simulink model "ASM_Traffic_MultiCore"  (R2026a)
settings: Solver=ode1  StartTime=SIM.tstart.v  StopTime=SIM.tend.v  FixedStep=SIM.StepSize.v
PostLoadFcn:
  | if any(exist('dsrtsu_mdlpostloadfcn', 'file') ~= 0), dsrtsu_mdlpostloadfcn('Execute', bdroot); end
  | try, asm_mdl_postloadfcn(bdroot, 'UpdateModel', 3600); catch, disp(lasterr); end,
InitFcn:
  | , if any(exist('rtifpga_mdlclblib', 'file') ~= 0), rtifpga_mdlclblib('Init', bdroot); end,
  | , if any(exist('dsmpb_private', 'file') ~= 0), dsmpb_private('dsmpb_mdlclblib', 'Init', bdroot); end,
model workspace (MAT data in the model file):
  asmReferencePath = [0 0.01 0.02 0.03 0.04 0.05 0.06 0.07 0.08 0.09 0.1 0.11 ... (350007 elements, 50001x7)]
  roadBounds : Simulink.Parameter (value not decoded)
  safetyAxes : Simulink.Parameter (value not decoded)
undefined symbols (not defined in the file): _to_, a0b2, ASM_BrakeHydraulics_DemoSystems, ASM_VehicleDynamics_DemoSystems, b98103fe8ad365046cd0, BrakeCircuit, controllerConfig, CPT, Crankshaft, DiscIntNeverNeededParam, dsmsi, FinalDriveAssembly, MDL, ModeSignals, mu, Pos_BrakePedal_Maneuver, rad, RefSignals, roadFamilyData, roadFamilyId, s_to_rpm, SIM, SoftECU, Suspension, Tire, Transmission
libraries: ASM_Traffic_lib x135, simulink x98, ASM_Utils_lib x77, ASM_VehicleDynamics_lib x70, ASM_Environment_lib x22, dsmpblib x20, dsmsilib x15, MDLD_Utils_lib x10, ASM_BrakeHydraulics_lib x3, sl_discontinuities x2
(part 25 of 65)

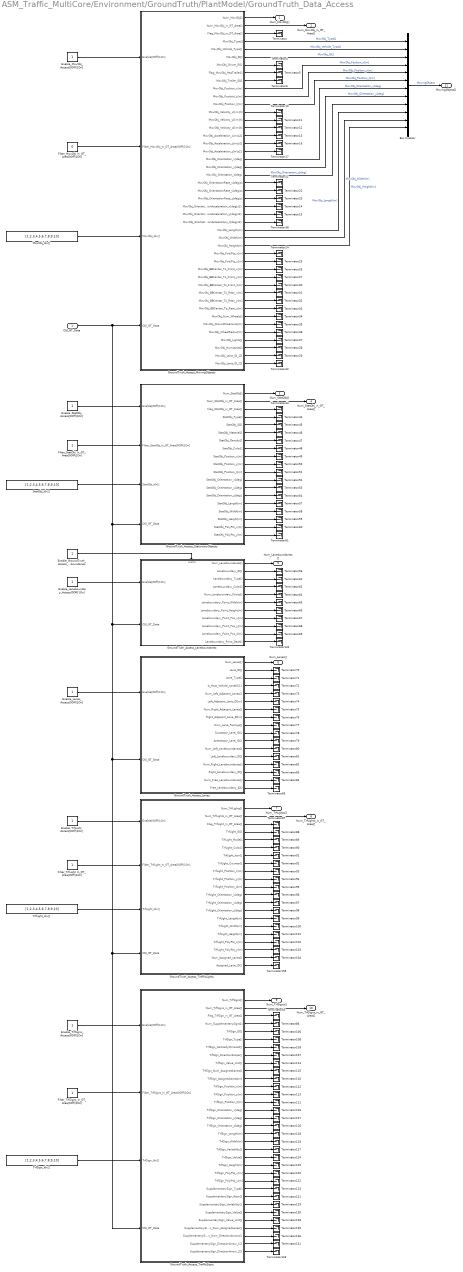
== system ASM_Traffic_MultiCore/Environment/GroundTruth/PlantModel/GroundTruth_Data_Access ==
  OSI_GT_Data : Inport
  Bus Creator : BusCreator  Inputs=12
  Enable_GroundTruth_Access_Laneboundaries : Constant
  Enable_Laneboundary_Access[0Off|1On] : Constant
  Enable_Lanes_Access[0Off|1On] : Constant
  Enable_MovObj_Access[0Off|1On] : Constant
  Enable_StatObj_Access[0Off|1On] : Constant
  Enable_TrfLight_Access[0Off|1On] : Constant
  Enable_TrfSigns_Access[0Off|1On] : Constant
  Filter_MovObj_In_GT_Area[0Off|1On] : Constant  Value=0
  Filter_StatObj_In_GT_Area[0Off|1On] : Constant
  Filter_TrfLight_In_GT_Area[0Off|1On] : Constant
  Filter_TrfSigns_In_GT_Area[0Off|1On] : Constant
  GroundTruth_Access_Laneboundaries : Subsystem
  GroundTruth_Access_Lanes : Subsystem
  GroundTruth_Access_MovingObjects : Subsystem
  GroundTruth_Access_StationaryObjects : Subsystem
  GroundTruth_Access_TrafficLights : Subsystem
  GroundTruth_Access_TrafficSigns : Subsystem
  MovObj_Idx[] : Constant  Value=[1,2,3,4,5,6,7,8,9,10]
  StatObj_Idx[] : Constant  Value=[1,2,3,4,5,6,7,8,9,10]
  Terminator{,4..6,10..17,21..38,42..133,135..136} (124 alike) : Terminator
  TrfLight_Idx[] : Constant  Value=[1,2,3,4,5,6,7,8,9,10]
  TrfSign_Idx[] : Constant  Value=[1,2,3,4,5,6,7,8,9,10]
  Num_MovObj[] : Outport  VectorParamsAs1DForOutWhenUnconnected=off
  Num_MovObj_in_GT_Area[] : Outport  Port=2  VectorParamsAs1DForOutWhenUnconnected=off
  Num_StatObj[] : Outport  Port=3  VectorParamsAs1DForOutWhenUnconnected=off
  Num_StatObj_in_GT_Area[] : Outport  Port=4  VectorParamsAs1DForOutWhenUnconnected=off
  Num_Laneboundaries[] : Outport  Port=5  VectorParamsAs1DForOutWhenUnconnected=off
  Num_Lanes[] : Outport  Port=6  VectorParamsAs1DForOutWhenUnconnected=off
  Num_TrfLights[] : Outport  Port=7  VectorParamsAs1DForOutWhenUnconnected=off
  Num_TrfLights_in_GT_Area[] : Outport  Port=8  VectorParamsAs1DForOutWhenUnconnected=off
  Num_TrfSigns[] : Outport  Port=9  VectorParamsAs1DForOutWhenUnconnected=off
  Num_TrfSigns_in_GT_Area[] : Outport  Port=10  VectorParamsAs1DForOutWhenUnconnected=off
  MovingObject[] : Outport  Port=11
  wires:
  Bus Creator/1 -> MovingObject[]/1  "MovingObject"
  GroundTruth_Access_Laneboundaries/11(Laneboundary_Point_Dash[]) -> Terminator132/1
  Enable_GroundTruth_Access_Laneboundaries/1 -> GroundTruth_Access_Laneboundaries/Enable
  GroundTruth_Access_MovingObjects/45(MovObj_Lane_ID_2[]) -> Terminator42/1
  GroundTruth_Access_MovingObjects/44(MovObj_Lane_ID_1[]) -> Terminator29/1
  GroundTruth_Access_MovingObjects/43(MovObj_NumLanes[]) -> Terminator28/1
  GroundTruth_Access_MovingObjects/42(MovObj_Lights[]) -> Terminator37/1
  GroundTruth_Access_MovingObjects/41(MovObj_WheelRadius[m]) -> Terminator36/1
  GroundTruth_Access_MovingObjects/40(MovObj_GroundClearance[m]) -> Terminator35/1
  GroundTruth_Access_MovingObjects/39(MovObj_Num_Wheels[]) -> Terminator34/1
  GroundTruth_Access_MovingObjects/38(MovObj_BBCenter_To_Rear_z[m]) -> Terminator33/1
  GroundTruth_Access_MovingObjects/37(MovObj_BBCenter_To_Rear_y[m]) -> Terminator32/1
  GroundTruth_Access_MovingObjects/36(MovObj_BBCenter_To_Rear_x[m]) -> Terminator31/1
  GroundTruth_Access_MovingObjects/35(MovObj_BBCenter_To_Front_z[m]) -> Terminator30/1
  GroundTruth_Access_MovingObjects/34(MovObj_BBCenter_To_Front_y[m]) -> Terminator27/1
  GroundTruth_Access_MovingObjects/33(MovObj_BBCenter_To_Front_x[m]) -> Terminator26/1
  GroundTruth_Access_MovingObjects/32(MovObj_PolyPts_y[m]) -> Terminator25/1
  GroundTruth_Access_MovingObjects/31(MovObj_PolyPts_x[m]) -> Terminator24/1
  GroundTruth_Access_MovingObjects/30(MovObj_Height[m]) -> Bus Creator/12  "MovObj_Height[m]"
  GroundTruth_Access_MovingObjects/29(MovObj_Width[m]) -> Bus Creator/11  "MovObj_Width[m]"
  GroundTruth_Access_MovingObjects/28(MovObj_Length[m]) -> Bus Creator/10  "MovObj_Length[m]"
  GroundTruth_Access_MovingObjects/27(MovObj_OrientationAcceleration_z[deg|s2]) -> Terminator38/1
  GroundTruth_Access_MovingObjects/26(MovObj_OrientationAcceleration_y[deg|s2]) -> Terminator15/1
  GroundTruth_Access_MovingObjects/25(MovObj_OrientationAcceleration_x[deg|s2]) -> Terminator14/1
  GroundTruth_Access_MovingObjects/24(MovObj_OrientationRate_z[deg|s]) -> Terminator23/1
  GroundTruth_Access_MovingObjects/23(MovObj_OrientationRate_y[deg|s]) -> Terminator22/1
  GroundTruth_Access_MovingObjects/22(MovObj_OrientationRate_x[deg|s]) -> Terminator21/1
  GroundTruth_Access_MovingObjects/21(MovObj_Orientation_z[deg]) -> Bus Creator/9  "MovObj_Orientation_z[deg]"
  GroundTruth_Access_MovingObjects/20(MovObj_Orientation_y[deg]) -> Bus Creator/8  "MovObj_Orientation_y[deg]"
  GroundTruth_Access_MovingObjects/19(MovObj_Orientation_x[deg]) -> Bus Creator/7  "MovObj_Orientation_x[deg]"
  GroundTruth_Access_MovingObjects/18(MovObj_Acceleration_z[m|s2]) -> Terminator17/1
  GroundTruth_Access_MovingObjects/17(MovObj_Acceleration_y[m|s2]) -> Terminator16/1
  GroundTruth_Access_MovingObjects/16(MovObj_Acceleration_x[m|s2]) -> Terminator13/1
  GroundTruth_Access_MovingObjects/15(MovObj_Velocity_z[km|h]) -> Terminator12/1
  GroundTruth_Access_MovingObjects/14(MovObj_Velocity_y[km|h]) -> Terminator11/1
  GroundTruth_Access_MovingObjects/13(MovObj_Velocity_x[km|h]) -> Terminator10/1
  GroundTruth_Access_MovingObjects/12(MovObj_Position_z[m]) -> Bus Creator/6  "MovObj_Position_z[m]"
  GroundTruth_Access_MovingObjects/11(MovObj_Position_y[m]) -> Bus Creator/5  "MovObj_Position_y[m]"
  GroundTruth_Access_MovingObjects/10(MovObj_Position_x[m]) -> Bus Creator/4  "MovObj_Position_x[m]"
  GroundTruth_Access_MovingObjects/9(MovObj_Trailer_ID[]) -> Terminator6/1
  GroundTruth_Access_MovingObjects/8(Flag_MovObj_HasTrailer[]) -> Terminator5/1
  GroundTruth_Access_MovingObjects/7(MovObj_Driver_ID[]) -> Terminator4/1
  GroundTruth_Access_MovingObjects/6(MovObj_ID[]) -> Bus Creator/3  "MovObj_ID[]"
  GroundTruth_Access_MovingObjects/5(MovObj_Vehicle_Type[]) -> Bus Creator/2  "MovObj_Vehicle_Type[]"
  GroundTruth_Access_MovingObjects/4(MovObj_Type[]) -> Bus Creator/1  "MovObj_Type[]"
  GroundTruth_Access_MovingObjects/3(Flag_MovObj_in_GT_Area[]) -> Terminator/1
  GroundTruth_Access_MovingObjects/2(Num_MovObj_in_GT_Area[]) -> Num_MovObj_in_GT_Area[]/1
  GroundTruth_Access_MovingObjects/1(Num_MovObj[]) -> Num_MovObj[]/1
  OSI_GT_Data/1 -> GroundTruth_Access_StationaryObjects/4(OSI_GT_Data), GroundTruth_Access_TrafficSigns/4(OSI_GT_Data), GroundTruth_Access_TrafficLights/4(OSI_GT_Data), GroundTruth_Access_Lanes/2(OSI_GT_Data), GroundTruth_Access_Laneboundaries/2(OSI_GT_Data), GroundTruth_Access_MovingObjects/4(OSI_GT_Data)
  MovObj_Idx[]/1 -> GroundTruth_Access_MovingObjects/3(MovObj_Idx[])
  Filter_MovObj_In_GT_Area[0Off|1On]/1 -> GroundTruth_Access_MovingObjects/2(Filter_MovObj_In_GT_Area[0Off|1On])
  Enable_MovObj_Access[0Off|1On]/1 -> GroundTruth_Access_MovingObjects/1(Enable[0Off|1On])
  GroundTruth_Access_StationaryObjects/2(Num_StatObj_in_GT_Area[]) -> Num_StatObj_in_GT_Area[]/1
  Enable_StatObj_Access[0Off|1On]/1 -> GroundTruth_Access_StationaryObjects/1(Enable[0Off|1On])
  Filter_StatObj_In_GT_Area[0Off|1On]/1 -> GroundTruth_Access_StationaryObjects/2(Filter_StatObj_In_GT_Area[0Off|1On])
  StatObj_Idx[]/1 -> GroundTruth_Access_StationaryObjects/3(StatObj_Idx[])
  GroundTruth_Access_Laneboundaries/1(Num_Laneboundaries[]) -> Num_Laneboundaries[]/1
  GroundTruth_Access_Laneboundaries/2(Laneboundary_ID[]) -> Terminator56/1
  GroundTruth_Access_Laneboundaries/3(Laneboundary_Type[]) -> Terminator62/1
  GroundTruth_Access_Laneboundaries/4(Laneboundary_Color[]) -> Terminator63/1
  GroundTruth_Access_Laneboundaries/5(Num_Laneboundary_Points[]) -> Terminator64/1
  GroundTruth_Access_Laneboundaries/6(Laneboundary_Point_Width[m]) -> Terminator65/1
  GroundTruth_Access_Laneboundaries/7(Laneboundary_Point_Height[m]) -> Terminator66/1
  GroundTruth_Access_Laneboundaries/8(Laneboundary_Point_Pos_x[m]) -> Terminator67/1
  GroundTruth_Access_Laneboundaries/9(Laneboundary_Point_Pos_y[m]) -> Terminator68/1
  GroundTruth_Access_Laneboundaries/10(Laneboundary_Point_Pos_z[m]) -> Terminator69/1
  Enable_Laneboundary_Access[0Off|1On]/1 -> GroundTruth_Access_Laneboundaries/1(Enable[0Off|1On])
  GroundTruth_Access_Lanes/1(Num_Lanes[]) -> Num_Lanes[]/1
  GroundTruth_Access_Lanes/2(Lane_ID[]) -> Terminator70/1
  GroundTruth_Access_Lanes/3(Lane_Type[]) -> Terminator71/1
  GroundTruth_Access_Lanes/4(Is_Host_Vehicle_Lane[0|1]) -> Terminator72/1
  GroundTruth_Access_Lanes/5(Num_Left_Adjacent_Lanes[]) -> Terminator73/1
  GroundTruth_Access_Lanes/6(Left_Adjacent_Lane_ID[m]) -> Terminator74/1
  GroundTruth_Access_Lanes/7(Num_Right_Adjacent_Lanes[]) -> Terminator75/1
  GroundTruth_Access_Lanes/8(Right_Adjacent_Lane_ID[m]) -> Terminator76/1
  GroundTruth_Access_Lanes/9(Num_Lane_Pairings[]) -> Terminator77/1
  GroundTruth_Access_Lanes/10(Successor_Lane_ID[]) -> Terminator78/1
  GroundTruth_Access_Lanes/11(Antecessor_Lane_ID[]) -> Terminator79/1
  GroundTruth_Access_Lanes/12(Num_Left_Laneboundaries[]) -> Terminator80/1
  GroundTruth_Access_Lanes/13(Left_Laneboundary_ID[]) -> Terminator81/1
  GroundTruth_Access_Lanes/14(Num_Right_Laneboundaries[]) -> Terminator82/1
  GroundTruth_Access_Lanes/15(Right_Laneboundary_ID[]) -> Terminator83/1
  GroundTruth_Access_Lanes/16(Num_Free_Laneboundaries[]) -> Terminator84/1
  GroundTruth_Access_Lanes/17(Free_Laneboundary_ID[]) -> Terminator85/1
  Enable_Lanes_Access[0Off|1On]/1 -> GroundTruth_Access_Lanes/1(Enable[0Off|1On])
  GroundTruth_Access_TrafficLights/2(Num_TrfLights_in_GT_Area[]) -> Num_TrfLights_in_GT_Area[]/1
  GroundTruth_Access_TrafficLights/1(Num_TrfLights[]) -> Num_TrfLights[]/1
  GroundTruth_Access_TrafficLights/3(Flag_TrfLight_in_GT_Area[]) -> Terminator87/1
  GroundTruth_Access_TrafficLights/4(TrfLight_ID[]) -> Terminator88/1
  GroundTruth_Access_TrafficLights/5(TrfLight_Mode[]) -> Terminator89/1
  GroundTruth_Access_TrafficLights/6(TrfLight_Color[]) -> Terminator90/1
  GroundTruth_Access_TrafficLights/7(TrfLight_Icon[]) -> Terminator91/1
  GroundTruth_Access_TrafficLights/8(TrfLight_Counter[]) -> Terminator92/1
  GroundTruth_Access_TrafficLights/9(TrfLight_Position_x[m]) -> Terminator93/1
  GroundTruth_Access_TrafficLights/10(TrfLight_Position_y[m]) -> Terminator94/1
  GroundTruth_Access_TrafficLights/11(TrfLight_Position_z[m]) -> Terminator95/1
  GroundTruth_Access_TrafficLights/12(TrfLight_Orientation_x[deg]) -> Terminator96/1
  GroundTruth_Access_TrafficLights/13(TrfLight_Orientation_y[deg]) -> Terminator97/1
  GroundTruth_Access_TrafficLights/14(TrfLight_Orientation_z[deg]) -> Terminator98/1
  GroundTruth_Access_TrafficLights/15(TrfLight_Length[m]) -> Terminator99/1
  GroundTruth_Access_TrafficLights/16(TrfLight_Width[m]) -> Terminator100/1
  GroundTruth_Access_TrafficLights/17(TrfLight_Height[m]) -> Terminator101/1
  GroundTruth_Access_TrafficLights/18(TrfLight_PolyPts_x[m]) -> Terminator102/1
  GroundTruth_Access_TrafficLights/19(TrfLight_PolyPts_y[m]) -> Terminator103/1
  GroundTruth_Access_TrafficLights/20(Num_Assigned_Lanes[]) -> Terminator104/1
  GroundTruth_Access_TrafficLights/21(Assigned_Lane_ID[]) -> Terminator105/1
  Enable_TrfLight_Access[0Off|1On]/1 -> GroundTruth_Access_TrafficLights/1(Enable[0Off|1On])
  Filter_TrfLight_In_GT_Area[0Off|1On]/1 -> GroundTruth_Access_TrafficLights/2(Filter_TrfLight_In_GT_Area[0Off|1On])
  TrfLight_Idx[]/1 -> GroundTruth_Access_TrafficLights/3(TrfLight_Idx[])
  GroundTruth_Access_TrafficSigns/3(Flag_TrfSign_in_GT_Area[]) -> Terminator55/1
  GroundTruth_Access_TrafficSigns/4(Num_SupplementarySigns[]) -> Terminator86/1
  GroundTruth_Access_TrafficSigns/5(TrfSign_ID[]) -> Terminator106/1
  GroundTruth_Access_TrafficSigns/6(TrfSign_Type[]) -> Terminator108/1
  GroundTruth_Access_TrafficSigns/7(TrfSign_VerticallyMirrored[]) -> Terminator109/1
  GroundTruth_Access_TrafficSigns/8(TrfSign_DirectionScope[]) -> Terminator107/1
  GroundTruth_Access_TrafficSigns/14(TrfSign_Position_z[m]) -> Terminator111/1
  GroundTruth_Access_TrafficSigns/13(TrfSign_Position_y[m]) -> Terminator113/1
  GroundTruth_Access_TrafficSigns/12(TrfSign_Position_x[m]) -> Terminator112/1
  GroundTruth_Access_TrafficSigns/11(TrfSign_AssignedLanes[m]) -> Terminator110/1
  GroundTruth_Access_TrafficSigns/10(TrfSign_Num_AssignedLanes[]) -> Terminator115/1
  GroundTruth_Access_TrafficSigns/9(TrfSign_Value_Unit[]) -> Terminator114/1
  GroundTruth_Access_TrafficSigns/21(TrfSign_Value[]) -> Terminator124/1
  GroundTruth_Access_TrafficSigns/22(TrfSign_Height[m]) -> Terminator125/1
  GroundTruth_Access_TrafficSigns/23(TrfSign_PolyPts_x[m]) -> Terminator120/1
  GroundTruth_Access_TrafficSigns/24(TrfSign_PolyPts_y[m]) -> Terminator122/1
  GroundTruth_Access_TrafficSigns/25(SupplementarySign_Type[]) -> Terminator123/1
  GroundTruth_Access_TrafficSigns/26(SupplementarySign_Actor[]) -> Terminator121/1
  GroundTruth_Access_TrafficSigns/20(TrfSign_Variability[]) -> Terminator117/1
  GroundTruth_Access_TrafficSigns/19(TrfSign_Width[m]) -> Terminator119/1
  GroundTruth_Access_TrafficSigns/18(TrfSign_Length[m]) -> Terminator118/1
  GroundTruth_Access_TrafficSigns/17(TrfSign_Orientation_z[deg]) -> Terminator116/1
  GroundTruth_Access_TrafficSigns/16(TrfSign_Orientation_y[deg]) -> Terminator127/1
  GroundTruth_Access_TrafficSigns/15(TrfSign_Orientation_x[deg]) -> Terminator126/1
  GroundTruth_Access_TrafficSigns/27(SupplementarySign_Variability[]) -> Terminator129/1
  GroundTruth_Access_TrafficSigns/28(SupplementarySign_Value[]) -> Terminator130/1
  GroundTruth_Access_TrafficSigns/29(SupplementarySign_Value_Unit[]) -> Terminator128/1
  GroundTruth_Access_TrafficSigns/33(SupplementarySign_DirectionArrow_2[]) -> Terminator133/1
  GroundTruth_Access_TrafficSigns/32(SupplementarySign_DirectionArrow_1[]) -> Terminator131/1
  GroundTruth_Access_TrafficSigns/31(SupplementarySign_Num_DirectionArrows[]) -> Terminator136/1
  GroundTruth_Access_TrafficSigns/30(SupplementarySign_Num_AssignedLanes[]) -> Terminator135/1
  Enable_TrfSigns_Access[0Off|1On]/1 -> GroundTruth_Access_TrafficSigns/1(Enable[0Off|1On])
  Filter_TrfSigns_In_GT_Area[0Off|1On]/1 -> GroundTruth_Access_TrafficSigns/2(Filter_TrfSigns_In_GT_Area[0Off|1On])
  TrfSign_Idx[]/1 -> GroundTruth_Access_TrafficSigns/3(TrfSign_Idx[])
  GroundTruth_Access_TrafficSigns/1(Num_TrfSigns[]) -> Num_TrfSigns[]/1
  GroundTruth_Access_TrafficSigns/2(Num_TrfSigns_in_GT_Area[]) -> Num_TrfSigns_in_GT_Area[]/1
  GroundTruth_Access_StationaryObjects/11(StatObj_Position_z[m]) -> Terminator51/1
  GroundTruth_Access_StationaryObjects/18(StatObj_PolyPts_x[m]) -> Terminator60/1
  GroundTruth_Access_StationaryObjects/4(StatObj_Type[]) -> Terminator44/1
  GroundTruth_Access_StationaryObjects/12(StatObj_Orientation_x[deg]) -> Terminator52/1
  GroundTruth_Access_StationaryObjects/15(StatObj_Length[m]) -> Terminator57/1
  GroundTruth_Access_StationaryObjects/14(StatObj_Orientation_z[deg]) -> Terminator54/1
  GroundTruth_Access_StationaryObjects/8(StatObj_Color[]) -> Terminator48/1
  GroundTruth_Access_StationaryObjects/3(Flag_StatObj_in_GT_Area[]) -> Terminator43/1
  GroundTruth_Access_StationaryObjects/10(StatObj_Position_y[m]) -> Terminator50/1
  GroundTruth_Access_StationaryObjects/7(StatObj_Density[]) -> Terminator47/1
  GroundTruth_Access_StationaryObjects/9(StatObj_Position_x[m]) -> Terminator49/1
  GroundTruth_Access_StationaryObjects/6(StatObj_Material[]) -> Terminator46/1
  GroundTruth_Access_StationaryObjects/13(StatObj_Orientation_y[deg]) -> Terminator53/1
  GroundTruth_Access_StationaryObjects/16(StatObj_Width[m]) -> Terminator58/1
  GroundTruth_Access_StationaryObjects/19(StatObj_PolyPts_y[m]) -> Terminator61/1
  GroundTruth_Access_StationaryObjects/17(StatObj_Height[m]) -> Terminator59/1
  GroundTruth_Access_StationaryObjects/5(StatObj_ID[]) -> Terminator45/1
  GroundTruth_Access_StationaryObjects/1(Num_StatObj[]) -> Num_StatObj[]/1

== system ASM_Traffic_MultiCore/Environment/GroundTruth/PlantModel/HostVehicle_Data_Access ==
  OSI_HV_Data : Inport
  Enable_HostVehicle_Data_Access[0Off|1On] : Constant
  HostVehicle_Data_Access : Subsystem
  Terminator{,1..23} (24 alike) : Terminator
  wires:
  HostVehicle_Data_Access/5(HV_Position_BB[x;y;z][m]) -> Terminator4/1
  HostVehicle_Data_Access/6(HV_Velocity_BB[x;y;z][m|s]) -> Terminator5/1
  HostVehicle_Data_Access/3(HV_ID[]) -> Terminator2/1
  HostVehicle_Data_Access/4(HV_Pos_BrakePedal[0_1]) -> Terminator3/1
  HostVehicle_Data_Access/2(Time_Stamp_Nanos[ns]) -> Terminator1/1
  Enable_HostVehicle_Data_Access[0Off|1On]/1 -> HostVehicle_Data_Access/1(Enable[0Off|1On])
  OSI_HV_Data/1 -> HostVehicle_Data_Access/2(OSI_HV_Data)
  HostVehicle_Data_Access/1(Time_Stamp_Seconds[s]) -> Terminator/1
  HostVehicle_Data_Access/7(HV_Acceleration_BB[x;y;z][m|s2]) -> Terminator6/1
  HostVehicle_Data_Access/8(HV_Orientation_BB[x;y;z][rad]) -> Terminator7/1
  HostVehicle_Data_Access/9(HV_Current_Curvature[1|m]) -> Terminator8/1
  HostVehicle_Data_Access/10(HV_Steering_Angle[rad]) -> Terminator9/1
  HostVehicle_Data_Access/11(HV_Steering_Angle_dt[rad|s]) -> Terminator10/1
  HostVehicle_Data_Access/12(HV_Steering_Torque[Nm]) -> Terminator11/1
  HostVehicle_Data_Access/13(HV_Pos_AccPedal[0_1]) -> Terminator12/1
  HostVehicle_Data_Access/14(HV_Pos_ClutchPedal[0_1]) -> Terminator13/1
  HostVehicle_Data_Access/15(HV_Gear[]) -> Terminator14/1
  HostVehicle_Data_Access/16(HV_Type_Engine[]) -> Terminator15/1
  HostVehicle_Data_Access/17(HV_n_Engine[rpm]) -> Terminator16/1
  HostVehicle_Data_Access/18(HV_Trq_Engine[Nm]) -> Terminator17/1
  HostVehicle_Data_Access/19(HV_Vehicle_Weight[kg]) -> Terminator18/1
  HostVehicle_Data_Access/20(HV_Vehicle_Operating_State[]) -> Terminator19/1
  HostVehicle_Data_Access/21(HV_WheelData_Axle_Idx[]) -> Terminator20/1
  HostVehicle_Data_Access/22(HV_WheelData_Wheel_Idx[]) -> Terminator21/1
  HostVehicle_Data_Access/23(HV_WheelData_Wheel_Speed[rad|s]) -> Terminator22/1
  HostVehicle_Data_Access/24(HV_WheelData_Wheel_Slip[]) -> Terminator23/1

== system ASM_Traffic_MultiCore/Environment/GroundTruth/PlantModel/ObjectDataStreams ==
  In : Inport
  Bus Selector14 : BusSelector  OutputSignals=DataStream_1[].DataStream_1[],DataStream_2[].DataStream_2[],DataStream_3[].DataStream_3[],DataStream_4[].DataStream_4[],DataStream_5[].DataStream_5[],DataStream_6[].DataStream_6[],DataStream_7[].DataStream_7[],DataStream_8[].DataStream_8[]
  Mux : Mux  Inputs=8
  Objects_DataStreams[] : Outport  VectorParamsAs1DForOutWhenUnconnected=off
  wires:
  Mux/1 -> Objects_DataStreams[]/1
  Bus Selector14/7 -> Mux/7  "<DataStream_7[]>"
  Bus Selector14/8 -> Mux/8  "<DataStream_8[]>"
  Bus Selector14/3 -> Mux/3  "<DataStream_3[]>"
  Bus Selector14/6 -> Mux/6  "<DataStream_6[]>"
  Bus Selector14/4 -> Mux/4  "<DataStream_4[]>"
  Bus Selector14/1 -> Mux/1  "<DataStream_1[]>"
  Bus Selector14/5 -> Mux/5  "<DataStream_5[]>"
  In/1 -> Bus Selector14/1
  Bus Selector14/2 -> Mux/2  "<DataStream_2[]>"

== system ASM_Traffic_MultiCore/Environment/GroundTruth/PlantModel/Running_Maneuver ==
  ManeuverState[] : Inport
  Brake : RelationalOperator  Operator===  OutDataTypeStr=boolean  InputSameDT=off
  Constant : Constant  Value=3
  Constant1 : Constant  Value=4
  Data Type Conversion : DataTypeConversion  OutDataTypeStr=double  SaturateOnIntegerOverflow=off  RndMeth=Floor
  Logical Operator : Logic  Operator=OR  AllPortsSameDT=off  OutDataTypeStr=boolean
  Run : RelationalOperator  Operator===  OutDataTypeStr=boolean  InputSameDT=off
  EnableRun[0Off|1On] : Outport  VectorParamsAs1DForOutWhenUnconnected=off
  wires:
  Run/1 -> Logical Operator/1
  ManeuverState[]/1 -> Brake/1, Run/1
  Constant1/1 -> Brake/2
  Logical Operator/1 -> Data Type Conversion/1
  Constant/1 -> Run/2
  Brake/1 -> Logical Operator/2
  Data Type Conversion/1 -> EnableRun[0Off|1On]/1

== system ASM_Traffic_MultiCore/Environment/GroundTruth/PlantModel/TrafficLight_Counter ==
  In : Inport
  Bus Selector14 : BusSelector  OutputSignals=TrafficLight_Counter_1[].TrafficLight_Counter_1[],TrafficLight_Counter_2.TrafficLight_Counter_2[],TrafficLight_Counter_3.TrafficLight_Counter_3[],TrafficLight_Counter_4[].TrafficLight_Counter_4[]
  Mux2 : Mux
  TrafficLight_Counter[] : Outport  VectorParamsAs1DForOutWhenUnconnected=off
  wires:
  Bus Selector14/1 -> Mux2/1  "<TrafficLight_Counter_1[]>"
  In/1 -> Bus Selector14/1
  Bus Selector14/3 -> Mux2/3  "<TrafficLight_Counter_3[]>"
  Bus Selector14/2 -> Mux2/2  "<TrafficLight_Counter_2[]>"
  Bus Selector14/4 -> Mux2/4  "<TrafficLight_Counter_4[]>"
  Mux2/1 -> TrafficLight_Counter[]/1

== system ASM_Traffic_MultiCore/Environment/GroundTruth/PlantModel/VehicleBasics ==
  In : Inport
  OSIGroundTruth : Inport  Port=2
  Bus Selector : BusSelector  OutputSignals=Interface_In.ExternalModel.m_TotalVehicle[kg],Interface_In.ExternalModel.State_StartButton[-2|-1|0|1|2|3]
  Bus Selector1 : BusSelector  OutputSignals=HostVehicle_Data_VehicleBasics[].Mode_OperatingState[1Stim|2Int],HostVehicle_Data_VehicleBasics[].Stim_OperatingState[]
  Multiport Switch : MultiPortSwitch  Inputs=2  SaturateOnIntegerOverflow=off  InputSameDT=off
  StartButton_Mapping : Subsystem
  m_TotalVehicle[kg] : Outport  VectorParamsAs1DForOutWhenUnconnected=off
  OperatingState[] : Outport  Port=2  VectorParamsAs1DForOutWhenUnconnected=off
  wires:
  Multiport Switch/1 -> OperatingState[]/1  "OperatingState[]"
  Bus Selector1/2 -> Multiport Switch/2  "<Stim_OperatingState[]>"
  Bus Selector1/1 -> Multiport Switch/1  "<Mode_OperatingState[1Stim|2Int]>"
  OSIGroundTruth/1 -> Bus Selector1/1
  In/1 -> Bus Selector/1
  Bus Selector/1 -> m_TotalVehicle[kg]/1  "<m_TotalVehicle[kg]>"
  Bus Selector/2 -> StartButton_Mapping/1(State_StartButton[-2|-1|0|1|2|3])  "<State_StartButton[-2|-1|0|1|2|3]>"
  StartButton_Mapping/1(OperatingState[]) -> Multiport Switch/3

== system ASM_Traffic_MultiCore/Environment/GroundTruth/PlantModel/VehicleBrakeSystem ==
  In : Inport
  Bus Selector25 : BusSelector  OutputSignals=Interface_In.ExternalModel.Pos_BrakePedal[%]
  Gain : Gain  Gain=1/100
  Pos_BrakePedal[0_1] : Outport
  wires:
  Bus Selector25/1 -> Gain/1  "<Pos_BrakePedal[%]>"
  In/1 -> Bus Selector25/1
  Gain/1 -> Pos_BrakePedal[0_1]/1

== system ASM_Traffic_MultiCore/Environment/GroundTruth/PlantModel/VehicleLocalization ==
  In : Inport
  Bus Selector : BusSelector  OutputSignals=Longitude[deg],Latitude[deg]
  Bus Selector10 : BusSelector  OutputSignals=Maneuver.Plant.ManeuverScheduler.Parameters.Object_Type_ID[]
  Bus Selector2 : BusSelector  OutputSignals=Interface_In.ExternalModel.Pos_Vehicle_CoorSys_E[x;y;z][m]
  Bus Selector22 : BusSelector  OutputSignals=Road.Plant.UserSignals_Customized
  Bus Selector3 : BusSelector  OutputSignals=Object_Properties_Box.PosVec_x_CenterPnt_Object[m],Object_Properties_Box.PosVec_y_CenterPnt_Object[m],Object_Properties_Box.PosVec_z_CenterPnt_Object[m]
  Bus Selector4 : BusSelector  OutputSignals=Interface_In.ExternalModel.Angle_Vehicle_CoorSys_E[x;y;z][deg]
  Bus Selector5 : BusSelector  OutputSignals=Traffic.Plant.ObjectParameters.TrafficObjects.TrafficObject_Type_Data[]
  COORDINATE_TRANSFORMATION_B_TO_A : ASM_Utils_lib/MatrixOperations/COORDINATE_TRANSFORMATION_B_TO_A  ASMLibrary2Check=ASM_Traffic_lib
  ChangeLabel : Subsystem
      mask Display: disp('')
  Demux : Demux  Outputs=3
  Demux1 : Demux  Outputs=3
  GPS_POSITION : ASM_Environment_lib/Environment/Road/GPS_POSITION  Tag=ASM_SUBCOMPONENT  ASMProperties=struct('Name','GPS_POSITION','Version','3.0','Library','ASM_Environment_lib')  ASMInstanceName=GPS_Position  ASMInstanceID=2
      settings: AttributesFormatString=Instance Name: %<ASMInstanceName>\nInstance ID: %<ASMInstanceID>
  Mux : Mux  Inputs=3
  OBJECT_PROPERTIES_BOX : ASM_Traffic_lib/Objects/OBJECT_PROPERTIES_BOX  ASMProperties=struct('Name','OBJECT_PROPERTIES_BOX','Version','2.0','Library','ASM_Traffic_lib')  ASMInstanceName=object_properties_box  ASMInstanceID=1
  Terminator : Terminator
  Terminator1 : Terminator
  Pos_Veh_BoundingBox_GPS[Long;Lat;Alt][deg;deg;m] : Outport
  wires:
  Bus Selector22/1 -> GPS_POSITION/1  "<UserSignals_Customized>"
  GPS_POSITION/1 -> Terminator/1
  GPS_POSITION/2 -> Bus Selector/1
  Bus Selector/1 -> Mux/1  "<Longitude[deg]>"
  Bus Selector/2 -> Mux/2  "<Latitude[deg]>"
  Mux/1 -> Pos_Veh_BoundingBox_GPS[Long;Lat;Alt][deg;deg;m]/1
  Bus Selector10/1 -> OBJECT_PROPERTIES_BOX/1  "<Object_Type_ID[]>"
  In/1 -> Bus Selector4/1, Bus Selector5/1, Bus Selector10/1, Bus Selector2/1, Bus Selector22/1
  Bus Selector5/1 -> OBJECT_PROPERTIES_BOX/2  "<TrafficObject_Type_Data[]>"
  OBJECT_PROPERTIES_BOX/1 -> Terminator1/1
  Bus Selector2/1 -> Demux/1  "<Pos_Vehicle_CoorSys_E[x;y;z][m]>"
  Demux/1 -> COORDINATE_TRANSFORMATION_B_TO_A/1
  Demux/2 -> COORDINATE_TRANSFORMATION_B_TO_A/2
  Demux/3 -> COORDINATE_TRANSFORMATION_B_TO_A/3
  Bus Selector3/2 -> COORDINATE_TRANSFORMATION_B_TO_A/5  "<PosVec_y_CenterPnt_Object[m]>"
  Bus Selector3/1 -> COORDINATE_TRANSFORMATION_B_TO_A/4  "<PosVec_x_CenterPnt_Object[m]>"
  Bus Selector3/3 -> COORDINATE_TRANSFORMATION_B_TO_A/6  "<PosVec_z_CenterPnt_Object[m]>"
  OBJECT_PROPERTIES_BOX/2 -> Bus Selector3/1
  Demux1/1 -> COORDINATE_TRANSFORMATION_B_TO_A/7
  Demux1/2 -> COORDINATE_TRANSFORMATION_B_TO_A/8
  Demux1/3 -> COORDINATE_TRANSFORMATION_B_TO_A/9
  COORDINATE_TRANSFORMATION_B_TO_A/3 -> ChangeLabel/1(In1)  "Pos_z_CoorSysE[m]"
  COORDINATE_TRANSFORMATION_B_TO_A/1 -> GPS_POSITION/2  "Pos_x_CoorSysE[m]"
  COORDINATE_TRANSFORMATION_B_TO_A/2 -> GPS_POSITION/3  "Pos_y_CoorSysE[m]"
  Bus Selector4/1 -> Demux1/1  "<Angle_Vehicle_CoorSys_E[x;y;z][deg]>"
  ChangeLabel/1(Out1) -> Mux/3  "Altitude[m]"

== system ASM_Traffic_MultiCore/Environment/GroundTruth/PlantModel/VehiclePowertrain ==
  In : Inport
  Bus Selector : BusSelector  OutputSignals=Interface_In.ExternalModel.Pos_AccPedal[%],Interface_In.ExternalModel.Pos_ClutchPedal[%],Interface_In.ExternalModel.Gear[],Interface_In.ExternalModel.n_Engine_1[rpm],Interface_In.ExternalModel.n_Engine_2[rpm],Interface_In.ExternalModel.Type_Engine_1[0Unkown|1Other|2Otto|3Diesel|4Electric],Interface_In.ExternalModel.Type_Engine_2[0Unkown|1Other|2Otto|3Diesel|4Electric],Interface_In.ExternalModel.Trq_Engine_1[Nm],Interface_In.ExternalModel.Trq_Engine_2[Nm]
  Gain : Gain  Gain=1/100
  Gain1 : Gain  Gain=1/100
  Mux : Mux  Inputs=2
  Mux1 : Mux  Inputs=2
  Mux2 : Mux  Inputs=2
  Pos_AccPedal[0_1] : Outport  VectorParamsAs1DForOutWhenUnconnected=off
  Pos_ClutchPedal[0_1] : Outport  Port=2  VectorParamsAs1DForOutWhenUnconnected=off
  Gear[] : Outport  Port=3  VectorParamsAs1DForOutWhenUnconnected=off
  n_Engine[rpm] : Outport  Port=4  VectorParamsAs1DForOutWhenUnconnected=off
  Type_Engine[0Unkown|1Other|2Otto|3Diesel|4Electric] : Outport  Port=5  VectorParamsAs1DForOutWhenUnconnected=off
  Trq_Engine[Nm] : Outport  Port=6  VectorParamsAs1DForOutWhenUnconnected=off
  wires:
  Bus Selector/3 -> Gear[]/1  "<Gear[]>"
  Bus Selector/4 -> Mux/1  "<n_Engine_1[rpm]>"
  Bus Selector/2 -> Gain1/1  "<Pos_ClutchPedal[%]>"
  In/1 -> Bus Selector/1
  Bus Selector/1 -> Gain/1  "<Pos_AccPedal[%]>"
  Mux/1 -> n_Engine[rpm]/1
  Bus Selector/5 -> Mux/2  "<n_Engine_2[rpm]>"
  Bus Selector/6 -> Mux1/1  "<Type_Engine_1[0Unkown|1Other|2Otto|3Diesel|4Electric]>"
  Bus Selector/7 -> Mux1/2  "<Type_Engine_2[0Unkown|1Other|2Otto|3Diesel|4Electric]>"
  Bus Selector/8 -> Mux2/1  "<Trq_Engine_1[Nm]>"
  Bus Selector/9 -> Mux2/2  "<Trq_Engine_2[Nm]>"
  Mux1/1 -> Type_Engine[0Unkown|1Other|2Otto|3Diesel|4Electric]/1
  Mux2/1 -> Trq_Engine[Nm]/1
  Gain/1 -> Pos_AccPedal[0_1]/1
  Gain1/1 -> Pos_ClutchPedal[0_1]/1

== system ASM_Traffic_MultiCore/Environment/GroundTruth/PlantModel/VehicleSteering ==
  In : Inport
  Bus Selector24 : BusSelector  OutputSignals=Interface_In.ExternalModel.Angle_SteeringWheel_SteeringSystem[deg],Interface_In.ExternalModel.Angle_SteeringWheel_dt_SteeringSystem[deg|s],Interface_In.ExternalModel.Trq_SteeringWheel_SteeringSystem[Nm]
  UnitConversion : ASM_Utils_lib/UnitConversion/UnitConversion  Selection=deg_to_rad
  UnitConversion1 : ASM_Utils_lib/UnitConversion/UnitConversion  Selection=deg_to_rad
  Angle_SteeringWheel_SteeringSystem[rad] : Outport  VectorParamsAs1DForOutWhenUnconnected=off
  Angle_SteeringWheel_dt_SteeringSystem[rad|s] : Outport  Port=2  VectorParamsAs1DForOutWhenUnconnected=off
  Trq_SteeringWheel_SteeringSystem[Nm] : Outport  Port=3  VectorParamsAs1DForOutWhenUnconnected=off
  wires:
  In/1 -> Bus Selector24/1
  Bus Selector24/1 -> UnitConversion/1  "<Angle_SteeringWheel_SteeringSystem[deg]>"
  Bus Selector24/2 -> UnitConversion1/1  "<Angle_SteeringWheel_dt_SteeringSystem[deg|s]>"
  Bus Selector24/3 -> Trq_SteeringWheel_SteeringSystem[Nm]/1  "<Trq_SteeringWheel_SteeringSystem[Nm]>"
  UnitConversion/1 -> Angle_SteeringWheel_SteeringSystem[rad]/1
  UnitConversion1/1 -> Angle_SteeringWheel_dt_SteeringSystem[rad|s]/1

== system ASM_Traffic_MultiCore/Environment/GroundTruth/PlantModel/VehicleWheels ==
  In : Inport
  OSIGroundTruth : Inport  Port=2
  Bus Selector1 : BusSelector  OutputSignals=HostVehicle_Data_VehicleWheels[].Axle_Idx[],HostVehicle_Data_VehicleWheels[].Wheel_Idx[]
  Bus Selector37 : BusSelector  OutputSignals=Interface_In.ExternalModel.omega_Wheel[rad|s],Interface_In.ExternalModel.Slip_x_Wheel[]
  Axle_Idx[] : Outport  VectorParamsAs1DForOutWhenUnconnected=off
  Wheel_Idx[] : Outport  Port=2  VectorParamsAs1DForOutWhenUnconnected=off
  omega_Wheel[rad|s] : Outport  Port=3  VectorParamsAs1DForOutWhenUnconnected=off
  Slip_x_Wheel[] : Outport  Port=4  VectorParamsAs1DForOutWhenUnconnected=off
  wires:
  In/1 -> Bus Selector37/1
  Bus Selector37/1 -> omega_Wheel[rad|s]/1  "<omega_Wheel[rad|s]>"
  Bus Selector37/2 -> Slip_x_Wheel[]/1  "<Slip_x_Wheel[]>"
  Bus Selector1/1 -> Axle_Idx[]/1  "<Axle_Idx[]>"
  Bus Selector1/2 -> Wheel_Idx[]/1  "<Wheel_Idx[]>"
  OSIGroundTruth/1 -> Bus Selector1/1

== system ASM_Traffic_MultiCore/Environment/GroundTruth/UserInterface/ASMSignalBus_Plant ==
  In : Inport
  Terminator_1 : Terminator
  tag scope: ASMBUS_Traffic_GroundTruth=global
  wires:
  In/1 -> [ASMBUS_Traffic_GroundTruth]
  [ASMBUS_Traffic_GroundTruth] -> Terminator_1/1

== system ASM_Traffic_MultiCore/Environment/GroundTruth/UserInterface/DISP_Plant ==
  In : Inport
  Bus Selector : BusSelector  OutputSignals=Control.Interface_Mode[0Off|1ObjOnly|2ObjAndLanes]
  Bus Selector1 : BusSelector  OutputSignals=Data_Access.Num_MovObj[],Data_Access.Num_MovObj_in_GT_Area[],Data_Access.Num_StatObj[],Data_Access.Num_StatObj_in_GT_Area[],Data_Access.Num_Laneboundaries[],Data_Access.Num_Lanes[],Data_Access.Num_TrfLights[],Data_Access.Num_TrfLights_in_GT_Area[],Data_Access.Num_TrfSigns[],Data_Access.Num_TrfSigns_in_GT_Area[]
  Bus Selector2 : BusSelector  OutputSignals=Data_Access.Num_MovObj[],Data_Access.Num_MovObj_in_GT_Area[],Data_Access.Num_StatObj[],Data_Access.Num_StatObj_in_GT_Area[],Data_Access.Num_Laneboundaries[],Data_Access.Num_Lanes[],Data_Access.Num_TrfLights[],Data_Access.Num_TrfLights_in_GT_Area[],Data_Access.Num_TrfSigns[],Data_Access.Num_TrfSigns_in_GT_Area[]
  Interface_Mode : Scope
      settings: TimeSpan=5  ActiveDisplayYMinimum=-0.375  ActiveDisplayYMaximum=3.375  DataLoggingMaxPoints=20000  DataLoggingDecimation=10  DataLoggingVariableName=ScopeData7
  Interface_Mode[0Off|1ObjOnly|2ObjAndLanes] : Subsystem
      mask Display: disp('')
  Interface_Mode_Disp : Display
  Lanes_Laneboundaries : Scope  NumInputPorts=2
      settings: TimeSpan=5  ActiveDisplayYMinimum=-1.25  ActiveDisplayYMaximum=11.25  DataLoggingMaxPoints=20000  DataLoggingDecimation=10  DataLoggingVariableName=ScopeData4
  MovObj : Scope  NumInputPorts=2
      settings: TimeSpan=5  ActiveDisplayYMinimum=-1.25  ActiveDisplayYMaximum=11.25  DataLoggingMaxPoints=20000  DataLoggingDecimation=10  DataLoggingVariableName=ScopeData2
  Num_Laneboundaries : Display
  Num_Laneboundaries[] : Subsystem
      mask Display: disp('')
  Num_Lanes : Display
  Num_Lanes[] : Subsystem
      mask Display: disp('')
  Num_MovObj : Display
  Num_MovObj[] : Subsystem
      mask Display: disp('')
  Num_MovObj_in_GT_Area : Display
  Num_MovObj_in_GT_Area[] : Subsystem
      mask Display: disp('')
  Num_StatObj : Display
  Num_StatObj[] : Subsystem
      mask Display: disp('')
  Num_StatObj_in_GT_Area : Display
  Num_StatObj_in_GT_Area[] : Subsystem
      mask Display: disp('')
  Num_TrfLights : Display
  Num_TrfLights[] : Subsystem
      mask Display: disp('')
  Num_TrfLights_in_GT_Area : Display
  Num_TrfLights_in_GT_Area[] : Subsystem
      mask Display: disp('')
  Num_TrfSigns : Display
  Num_TrfSigns[] : Subsystem
      mask Display: disp('')
  Num_TrfSigns_in_GT_Area : Display
  Num_TrfSigns_in_GT_Area[] : Subsystem
      mask Display: disp('')
  StatObj : Scope  NumInputPorts=2
      settings: TimeSpan=5  ActiveDisplayYMinimum=-3  ActiveDisplayYMaximum=27  DataLoggingMaxPoints=20000  DataLoggingDecimation=10  DataLoggingVariableName=ScopeData3
  TrfLights : Scope  NumInputPorts=2
      settings: TimeSpan=5  ActiveDisplayYMinimum=-1  ActiveDisplayYMaximum=1  DataLoggingMaxPoints=20000  DataLoggingDecimation=10  DataLoggingVariableName=ScopeData5
  TrfSigns : Scope  NumInputPorts=2
      settings: TimeSpan=5  ActiveDisplayYMinimum=-1.5  ActiveDisplayYMaximum=13.5  DataLoggingMaxPoints=20000  DataLoggingDecimation=10  DataLoggingVariableName=ScopeData6
  wires:
  In/1 -> Bus Selector2/1, Bus Selector1/1, Bus Selector/1
  Bus Selector/1 -> Interface_Mode[0Off|1ObjOnly|2ObjAndLanes]/1(In1)  "<Interface_Mode[0Off|1ObjOnly|2ObjAndLanes]>"
  Bus Selector1/1 -> Num_MovObj[]/1(In1)  "<Num_MovObj[]>"
  Bus Selector1/2 -> Num_MovObj_in_GT_Area[]/1(In1)  "<Num_MovObj_in_GT_Area[]>"
  Bus Selector1/3 -> Num_StatObj[]/1(In1)  "<Num_StatObj[]>"
  Bus Selector1/4 -> Num_StatObj_in_GT_Area[]/1(In1)  "<Num_StatObj_in_GT_Area[]>"
  Bus Selector1/5 -> Num_Laneboundaries[]/1(In1)  "<Num_Laneboundaries[]>"
  Bus Selector1/6 -> Num_Lanes[]/1(In1)  "<Num_Lanes[]>"
  Bus Selector1/7 -> Num_TrfLights[]/1(In1)  "<Num_TrfLights[]>"
  Bus Selector1/8 -> Num_TrfLights_in_GT_Area[]/1(In1)  "<Num_TrfLights_in_GT_Area[]>"
  Bus Selector1/9 -> Num_TrfSigns[]/1(In1)  "<Num_TrfSigns[]>"
  Bus Selector1/10 -> Num_TrfSigns_in_GT_Area[]/1(In1)  "<Num_TrfSigns_in_GT_Area[]>"
  Num_MovObj[]/1(Out1) -> MovObj/1  "Num_MovObj[]"
  Num_MovObj_in_GT_Area[]/1(Out1) -> MovObj/2  "Num_MovObj_in_GT_Area[]"
  Interface_Mode[0Off|1ObjOnly|2ObjAndLanes]/1(Out1) -> Interface_Mode_Disp/1, Interface_Mode/1  "Interface_Mode[0Off|1ObjOnly|2ObjAndLanes]"
  Num_StatObj[]/1(Out1) -> StatObj/1  "Num_StatObj[]"
  Num_StatObj_in_GT_Area[]/1(Out1) -> StatObj/2  "Num_StatObj_in_GT_Area[]"
  Num_Laneboundaries[]/1(Out1) -> Lanes_Laneboundaries/1  "Num_Laneboundaries[]"
  Num_Lanes[]/1(Out1) -> Lanes_Laneboundaries/2  "Num_Lanes[]"
  Num_TrfLights[]/1(Out1) -> TrfLights/1  "Num_TrfLights[]"
  Num_TrfLights_in_GT_Area[]/1(Out1) -> TrfLights/2  "Num_TrfLights_in_GT_Area[]"
  Num_TrfSigns[]/1(Out1) -> TrfSigns/1  "Num_TrfSigns[]"
  Num_TrfSigns_in_GT_Area[]/1(Out1) -> TrfSigns/2  "Num_TrfSigns_in_GT_Area[]"
  Bus Selector2/1 -> Num_MovObj/1  "<Num_MovObj[]>"
  Bus Selector2/2 -> Num_MovObj_in_GT_Area/1  "<Num_MovObj_in_GT_Area[]>"
  Bus Selector2/3 -> Num_StatObj/1  "<Num_StatObj[]>"
  Bus Selector2/4 -> Num_StatObj_in_GT_Area/1  "<Num_StatObj_in_GT_Area[]>"
  Bus Selector2/5 -> Num_Laneboundaries/1  "<Num_Laneboundaries[]>"
  Bus Selector2/6 -> Num_Lanes/1  "<Num_Lanes[]>"
  Bus Selector2/7 -> Num_TrfLights/1  "<Num_TrfLights[]>"
  Bus Selector2/8 -> Num_TrfLights_in_GT_Area/1  "<Num_TrfLights_in_GT_Area[]>"
  Bus Selector2/9 -> Num_TrfSigns/1  "<Num_TrfSigns[]>"
  Bus Selector2/10 -> Num_TrfSigns_in_GT_Area/1  "<Num_TrfSigns_in_GT_Area[]>"

== system ASM_Traffic_MultiCore/Environment/GroundTruth/UserInterface/PAR_Plant ==
  Interface_In : Inport
  In : Inport  Port=2
  Bus Creator : BusCreator  Inputs=1
  Bus Creator1 : BusCreator  Inputs=9
  Country_Code[] : Constant  Tag=AD:ASM_Sw_SpeedLimit_Source[1Manual|2RoadScenery]
  Ego_Vehicle : Subsystem
  Enable_HostVehicle_Data[0Off|1On] : Constant  Tag=AD:ASM_Sw_SpeedLimit_Source[1Manual|2RoadScenery]
  Environmental_Conditions : Subsystem
  Fellow_Vehicles : Subsystem
  HostVehicle_Data_AutomatedDrivingFunction : Subsystem
  HostVehicle_Data_VehicleBasics : Subsystem
  HostVehicle_Data_VehicleWheels : Subsystem
  Terminator1 : Terminator
  TrafficLight_Counter : Subsystem
  Out : Outport  VectorParamsAs1DForOutWhenUnconnected=off
  wires:
  In/1 -> Terminator1/1
  Bus Creator/1 -> Out/1  "UserInterface"
  Bus Creator1/1 -> Bus Creator/1  "OSIGroundTruth"
  Enable_HostVehicle_Data[0Off|1On]/1 -> Bus Creator1/6  "Enable_HostVehicle_Data[0Off|1On]"
  HostVehicle_Data_VehicleWheels/1(HostVehicle_Data_VehicleWheels[]) -> Bus Creator1/7
  Ego_Vehicle/1(Ego_Vehicle[]) -> Bus Creator1/2
  Country_Code[]/1 -> Bus Creator1/1  "Country_Code[]"
  Fellow_Vehicles/1(Fellow_Vehicles[]) -> Bus Creator1/3
  Interface_In/1 -> HostVehicle_Data_AutomatedDrivingFunction/1(Interface_In), Fellow_Vehicles/1(Interface_In), Ego_Vehicle/1(Interface_In)
  Environmental_Conditions/1(Environmental_Conditions[]) -> Bus Creator1/4
  TrafficLight_Counter/1(TrafficLight_Counter[]) -> Bus Creator1/5
  HostVehicle_Data_AutomatedDrivingFunction/1(HostVehicle_Data_AutomatedDrivingFunction[]) -> Bus Creator1/9
  HostVehicle_Data_VehicleBasics/1(HostVehicle_Data_VehicleBasics[]) -> Bus Creator1/8

== system ASM_Traffic_MultiCore/Environment/Interface_In/ModelSignals/ACC_State[1OFF|2Standby|3ON]_ ==
  In1 : Inport
  DummyGain : Gain  SaturateOnIntegerOverflow=on  OutDataTypeStr=Inherit: Same as input  ParamDataTypeStr=Inherit: Same as input
  Out1 : Outport  VectorParamsAs1DForOutWhenUnconnected=off
  wires:
  DummyGain/1 -> Out1/1
  In1/1 -> DummyGain/1

== system ASM_Traffic_MultiCore/Environment/Interface_In/ModelSignals/AEB[0|1]_ ==
  In1 : Inport
  Gain : Gain  SaturateOnIntegerOverflow=on  OutDataTypeStr=Inherit: Same as input  ParamDataTypeStr=Inherit: Same as input
  Out1 : Outport  VectorParamsAs1DForOutWhenUnconnected=off
  wires:
  Gain/1 -> Out1/1
  In1/1 -> Gain/1

== system ASM_Traffic_MultiCore/Environment/Interface_In/ModelSignals/Active_CP_VehDyn_Trailer[]_ ==
  In1 : Inport
  Gain : Gain  SaturateOnIntegerOverflow=on  OutDataTypeStr=Inherit: Same as input  ParamDataTypeStr=Inherit: Same as input
  Out1 : Outport  VectorParamsAs1DForOutWhenUnconnected=off
  wires:
  In1/1 -> Gain/1
  Gain/1 -> Out1/1

== system ASM_Traffic_MultiCore/Environment/Interface_In/ModelSignals/Angle_SteeringWheel[deg]_ ==
  In1 : Inport
  DummyGain : Gain  SaturateOnIntegerOverflow=on  OutDataTypeStr=Inherit: Same as input  ParamDataTypeStr=Inherit: Same as input
  Out1 : Outport  VectorParamsAs1DForOutWhenUnconnected=off
  wires:
  DummyGain/1 -> Out1/1
  In1/1 -> DummyGain/1

== system ASM_Traffic_MultiCore/Environment/Interface_In/ModelSignals/Angle_SteeringWheel_SteeringSystem[deg]_ ==
  In1 : Inport
  Gain : Gain  SaturateOnIntegerOverflow=on  OutDataTypeStr=Inherit: Same as input  ParamDataTypeStr=Inherit: Same as input
  Out1 : Outport  VectorParamsAs1DForOutWhenUnconnected=off
  wires:
  Gain/1 -> Out1/1
  In1/1 -> Gain/1

== system ASM_Traffic_MultiCore/Environment/Interface_In/ModelSignals/Angle_SteeringWheel_dt_SteeringSystem[deg|s]_ ==
  In1 : Inport
  Gain : Gain  SaturateOnIntegerOverflow=on  OutDataTypeStr=Inherit: Same as input  ParamDataTypeStr=Inherit: Same as input
  Out1 : Outport  VectorParamsAs1DForOutWhenUnconnected=off
  wires:
  Gain/1 -> Out1/1
  In1/1 -> Gain/1

== system ASM_Traffic_MultiCore/Environment/Interface_In/ModelSignals/Angle_Vehicle_CoorSys_E[x;y;z][deg]_ ==
  In1 : Inport
  Gain : Gain  SaturateOnIntegerOverflow=on  OutDataTypeStr=Inherit: Same as input  ParamDataTypeStr=Inherit: Same as input
  Out1 : Outport  VectorParamsAs1DForOutWhenUnconnected=off
  wires:
  Gain/1 -> Out1/1
  In1/1 -> Gain/1

== system ASM_Traffic_MultiCore/Environment/Interface_In/ModelSignals/Coef_RollingRes[FL;FR;RL;RR][]_ ==
  In1 : Inport
  Gain : Gain  SaturateOnIntegerOverflow=on  OutDataTypeStr=Inherit: Same as input  ParamDataTypeStr=Inherit: Same as input
  Out1 : Outport  VectorParamsAs1DForOutWhenUnconnected=off
  wires:
  Gain/1 -> Out1/1
  In1/1 -> Gain/1

== system ASM_Traffic_MultiCore/Environment/Interface_In/ModelSignals/Coef_RollingRes_Mean[]_ ==
  In1 : Inport
  Gain : Gain  SaturateOnIntegerOverflow=on  OutDataTypeStr=Inherit: Same as input  ParamDataTypeStr=Inherit: Same as input
  Out1 : Outport  VectorParamsAs1DForOutWhenUnconnected=off
  wires:
  In1/1 -> Gain/1
  Gain/1 -> Out1/1

== system ASM_Traffic_MultiCore/Environment/Interface_In/ModelSignals/Const_r_unloaded_Tire_Mean[m]_ ==
  In1 : Inport
  Gain : Gain  SaturateOnIntegerOverflow=on  OutDataTypeStr=Inherit: Same as input  ParamDataTypeStr=Inherit: Same as input
  Out1 : Outport  VectorParamsAs1DForOutWhenUnconnected=off
  wires:
  In1/1 -> Gain/1
  Gain/1 -> Out1/1

== system ASM_Traffic_MultiCore/Environment/Interface_In/ModelSignals/CorneringStiffness[FL;FR;RL;RR][N]_ ==
  In1 : Inport
  Gain : Gain  SaturateOnIntegerOverflow=on  OutDataTypeStr=Inherit: Same as input  ParamDataTypeStr=Inherit: Same as input
  Out1 : Outport  VectorParamsAs1DForOutWhenUnconnected=off
  wires:
  Gain/1 -> Out1/1
  In1/1 -> Gain/1

== system ASM_Traffic_MultiCore/Environment/Interface_In/ModelSignals/Driver_Override_ACC_Active[0Off|1On]_ ==
  In1 : Inport
  DummyGain : Gain  SaturateOnIntegerOverflow=on  OutDataTypeStr=Inherit: Same as input  ParamDataTypeStr=Inherit: Same as input
  Out1 : Outport  VectorParamsAs1DForOutWhenUnconnected=off
  wires:
  DummyGain/1 -> Out1/1
  In1/1 -> DummyGain/1

== system ASM_Traffic_MultiCore/Environment/Interface_In/ModelSignals/Driver_Override_ACC_Reason[0NoOverride|1BrakePedal|2AccPedal]_ ==
  In1 : Inport
  DummyGain : Gain  SaturateOnIntegerOverflow=on  OutDataTypeStr=Inherit: Same as input  ParamDataTypeStr=Inherit: Same as input
  Out1 : Outport  VectorParamsAs1DForOutWhenUnconnected=off
  wires:
  DummyGain/1 -> Out1/1
  In1/1 -> DummyGain/1

== system ASM_Traffic_MultiCore/Environment/Interface_In/ModelSignals/FCW[0|1]_ ==
  In1 : Inport
  Gain : Gain  SaturateOnIntegerOverflow=on  OutDataTypeStr=Inherit: Same as input  ParamDataTypeStr=Inherit: Same as input
  Out1 : Outport  VectorParamsAs1DForOutWhenUnconnected=off
  wires:
  Gain/1 -> Out1/1
  In1/1 -> Gain/1

== system ASM_Traffic_MultiCore/Environment/Interface_In/ModelSignals/Gear[]_ ==
  In1 : Inport
  DummyGain : Gain  SaturateOnIntegerOverflow=on  OutDataTypeStr=Inherit: Same as input  ParamDataTypeStr=Inherit: Same as input
  Out1 : Outport  VectorParamsAs1DForOutWhenUnconnected=off
  wires:
  In1/1 -> DummyGain/1
  DummyGain/1 -> Out1/1

== system ASM_Traffic_MultiCore/Environment/Interface_In/ModelSignals/Mode_Drivetrain[1|2|3|4|5]_ ==
  In1 : Inport
  Gain : Gain  SaturateOnIntegerOverflow=on  OutDataTypeStr=Inherit: Same as input  ParamDataTypeStr=Inherit: Same as input
  Out1 : Outport  VectorParamsAs1DForOutWhenUnconnected=off
  wires:
  In1/1 -> Gain/1
  Gain/1 -> Out1/1

== system ASM_Traffic_MultiCore/Environment/Interface_In/ModelSignals/Mode_Transmission[1Manual|2Automatic]_ ==
  In1 : Inport
  Gain : Gain  SaturateOnIntegerOverflow=on  OutDataTypeStr=Inherit: Same as input  ParamDataTypeStr=Inherit: Same as input
  Out1 : Outport  VectorParamsAs1DForOutWhenUnconnected=off
  wires:
  In1/1 -> Gain/1
  Gain/1 -> Out1/1

== system ASM_Traffic_MultiCore/Environment/Interface_In/ModelSignals/Pos_AccPedal[%]_ ==
  In1 : Inport
  DummyGain : Gain  SaturateOnIntegerOverflow=on  OutDataTypeStr=Inherit: Same as input  ParamDataTypeStr=Inherit: Same as input
  Out1 : Outport  VectorParamsAs1DForOutWhenUnconnected=off
  wires:
  In1/1 -> DummyGain/1
  DummyGain/1 -> Out1/1

== system ASM_Traffic_MultiCore/Environment/Interface_In/ModelSignals/Pos_BrakePedal[%]_ ==
  In1 : Inport
  DummyGain : Gain  SaturateOnIntegerOverflow=on  OutDataTypeStr=Inherit: Same as input  ParamDataTypeStr=Inherit: Same as input
  Out1 : Outport  VectorParamsAs1DForOutWhenUnconnected=off
  wires:
  In1/1 -> DummyGain/1
  DummyGain/1 -> Out1/1

== system ASM_Traffic_MultiCore/Environment/Interface_In/ModelSignals/Pos_CP_FL2_Trailer_CoorSys_E[x;y][m]_ ==
  In1 : Inport
  Gain : Gain  SaturateOnIntegerOverflow=on  OutDataTypeStr=Inherit: Same as input  ParamDataTypeStr=Inherit: Same as input
  Out1 : Outport  VectorParamsAs1DForOutWhenUnconnected=off
  wires:
  Gain/1 -> Out1/1
  In1/1 -> Gain/1

== system ASM_Traffic_MultiCore/Environment/Interface_In/ModelSignals/Pos_CP_FL_CoorSys_E[x;y][m]_ ==
  In1 : Inport
  Gain : Gain  SaturateOnIntegerOverflow=on  OutDataTypeStr=Inherit: Same as input  ParamDataTypeStr=Inherit: Same as input
  Out1 : Outport  VectorParamsAs1DForOutWhenUnconnected=off
  wires:
  Gain/1 -> Out1/1
  In1/1 -> Gain/1

== system ASM_Traffic_MultiCore/Environment/Interface_In/ModelSignals/Pos_CP_FL_Trailer_CoorSys_E[x;y][m]_ ==
  In1 : Inport
  Gain : Gain  SaturateOnIntegerOverflow=on  OutDataTypeStr=Inherit: Same as input  ParamDataTypeStr=Inherit: Same as input
  Out1 : Outport  VectorParamsAs1DForOutWhenUnconnected=off
  wires:
  Gain/1 -> Out1/1
  In1/1 -> Gain/1

== system ASM_Traffic_MultiCore/Environment/Interface_In/ModelSignals/Pos_CP_FR2_Trailer_CoorSys_E[x;y][m]_ ==
  In1 : Inport
  Gain : Gain  SaturateOnIntegerOverflow=on  OutDataTypeStr=Inherit: Same as input  ParamDataTypeStr=Inherit: Same as input
  Out1 : Outport  VectorParamsAs1DForOutWhenUnconnected=off
  wires:
  Gain/1 -> Out1/1
  In1/1 -> Gain/1

== system ASM_Traffic_MultiCore/Environment/Interface_In/ModelSignals/Pos_CP_FR_CoorSys_E[x;y][m]_ ==
  In1 : Inport
  Gain : Gain  SaturateOnIntegerOverflow=on  OutDataTypeStr=Inherit: Same as input  ParamDataTypeStr=Inherit: Same as input
  Out1 : Outport  VectorParamsAs1DForOutWhenUnconnected=off
  wires:
  In1/1 -> Gain/1
  Gain/1 -> Out1/1

== system ASM_Traffic_MultiCore/Environment/Interface_In/ModelSignals/Pos_CP_FR_Trailer_CoorSys_E[x;y][m]_ ==
  In1 : Inport
  Gain : Gain  SaturateOnIntegerOverflow=on  OutDataTypeStr=Inherit: Same as input  ParamDataTypeStr=Inherit: Same as input
  Out1 : Outport  VectorParamsAs1DForOutWhenUnconnected=off
  wires:
  Gain/1 -> Out1/1
  In1/1 -> Gain/1

== system ASM_Traffic_MultiCore/Environment/Interface_In/ModelSignals/Pos_CP_Front_CoorSys_E[x;y][m]_ ==
  In1 : Inport
  Gain : Gain  SaturateOnIntegerOverflow=on  OutDataTypeStr=Inherit: Same as input  ParamDataTypeStr=Inherit: Same as input
  Out1 : Outport  VectorParamsAs1DForOutWhenUnconnected=off
  wires:
  In1/1 -> Gain/1
  Gain/1 -> Out1/1

== system ASM_Traffic_MultiCore/Environment/Interface_In/ModelSignals/Pos_CP_R2L2_CoorSys_E[x;y][m]_ ==
  In1 : Inport
  Gain : Gain  SaturateOnIntegerOverflow=on  OutDataTypeStr=Inherit: Same as input  ParamDataTypeStr=Inherit: Same as input
  Out1 : Outport  VectorParamsAs1DForOutWhenUnconnected=off
  wires:
  In1/1 -> Gain/1
  Gain/1 -> Out1/1

== system ASM_Traffic_MultiCore/Environment/Interface_In/ModelSignals/Pos_CP_R2L2_Trailer_CoorSys_E[x;y][m]_ ==
  In1 : Inport
  Gain : Gain  SaturateOnIntegerOverflow=on  OutDataTypeStr=Inherit: Same as input  ParamDataTypeStr=Inherit: Same as input
  Out1 : Outport  VectorParamsAs1DForOutWhenUnconnected=off
  wires:
  Gain/1 -> Out1/1
  In1/1 -> Gain/1

== system ASM_Traffic_MultiCore/Environment/Interface_In/ModelSignals/Pos_CP_R2L_CoorSys_E[x;y][m]_ ==
  In1 : Inport
  Gain : Gain  SaturateOnIntegerOverflow=on  OutDataTypeStr=Inherit: Same as input  ParamDataTypeStr=Inherit: Same as input
  Out1 : Outport  VectorParamsAs1DForOutWhenUnconnected=off
  wires:
  Gain/1 -> Out1/1
  In1/1 -> Gain/1

== system ASM_Traffic_MultiCore/Environment/Interface_In/ModelSignals/Pos_CP_R2L_Trailer_CoorSys_E[x;y][m]_ ==
  In1 : Inport
  Gain : Gain  SaturateOnIntegerOverflow=on  OutDataTypeStr=Inherit: Same as input  ParamDataTypeStr=Inherit: Same as input
  Out1 : Outport  VectorParamsAs1DForOutWhenUnconnected=off
  wires:
  Gain/1 -> Out1/1
  In1/1 -> Gain/1

== system ASM_Traffic_MultiCore/Environment/Interface_In/ModelSignals/Pos_CP_R2R2_CoorSys_E[x;y][m]_ ==
  In1 : Inport
  Gain : Gain  SaturateOnIntegerOverflow=on  OutDataTypeStr=Inherit: Same as input  ParamDataTypeStr=Inherit: Same as input
  Out1 : Outport  VectorParamsAs1DForOutWhenUnconnected=off
  wires:
  In1/1 -> Gain/1
  Gain/1 -> Out1/1
